simulink model "CHB_inverter_v2"  (R2025a)
settings: Solver=FixedStepDiscrete  StartTime=0.0  StopTime=T_stop  FixedStep=Ts  RelTol=1e-3
values from neighbouring files (symbols this model uses):
  Ts = Ts_pwr    (= 1e-06)    [init_microgrid.m]
  Vdc = sm(Vdc,100)    [make_figures.m]
undefined symbols (not defined in the file or in its folder): Cf, Lf, Rd, RLf, Rload
libraries: spsSeriesRLCBranchLib x3, spsUniversalBridgeLib x2, spsVoltageMeasurementLib x2, spsDCVoltageSourceLib x2, spsGroundLib x1, spsCurrentMeasurementLib x1, spspowerguiLib x1
settings Model: Creator=msssr  LastModifiedBy=msssr
settings DataIOCC: SignalLogging=off

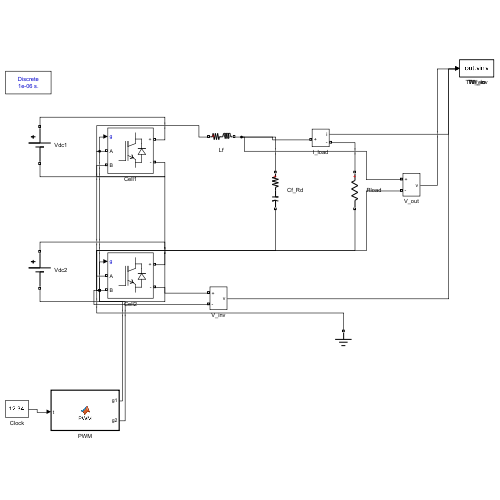
[thumbnail: Simulink's stored preview of the top-level diagram]
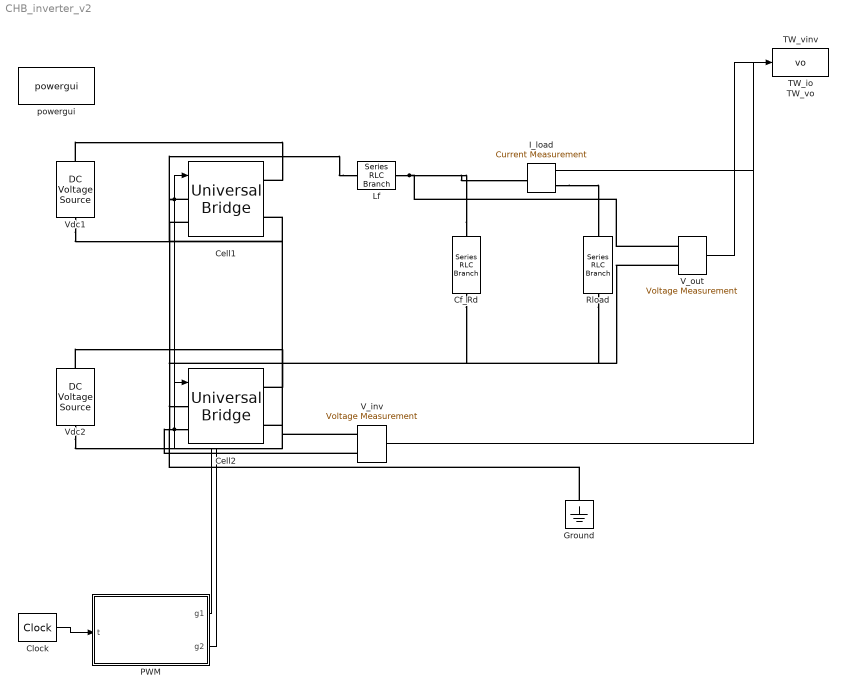
== system CHB_inverter_v2 ==
  Cell1 : spsUniversalBridgeLib/Universal Bridge  Arms=2  SnubberResistance=1e5  SnubberCapacitance=inf  Device=IGBT / Diodes  Ron=1e-3  Lon=0  ForwardVoltages="[  0  0  ]"  ForwardVoltage=0  GTOparameters=[ 10e-6 , 20e-6 ]  IGBTparameters=[ 1e-6 , 2e-6 ]  Measurements=None  Measurements_2=None  converterType=Rectifier
  Cell2 : spsUniversalBridgeLib/Universal Bridge  Arms=2  SnubberResistance=1e5  SnubberCapacitance=inf  Device=IGBT / Diodes  Ron=1e-3  Lon=0  ForwardVoltages="[  0  0  ]"  ForwardVoltage=0  GTOparameters=[ 10e-6 , 20e-6 ]  IGBTparameters=[ 1e-6 , 2e-6 ]  Measurements=None  Measurements_2=None  converterType=Rectifier
  Cf_Rd : spsSeriesRLCBranchLib/Series RLC Branch  LConnTagsString=__new0  RConnTagsString=__new0  BranchType=RC  Resistance=max(Rd,1e-6)  Inductance=1e-3  SetiL0=off  InitialCurrent=0  Capacitance=Cf  Setx0=off  InitialVoltage=0  Measurements=None
  Clock : DigitalClock  SampleTime=Ts
  Ground : spsGroundLib/Ground  LConnTagsString=a
  I_load : spsCurrentMeasurementLib/Current Measurement  PhasorSimulation=off  OutputType=Complex  PSBequivalent=0
  Lf : spsSeriesRLCBranchLib/Series RLC Branch  LConnTagsString=__new0  RConnTagsString=__new0  BranchType=RL  Resistance=RLf  Inductance=Lf  SetiL0=off  InitialCurrent=0  Capacitance=1e-6  Setx0=off  InitialVoltage=0  Measurements=None
  PWM : MATLAB Function  TreatAsAtomicUnit=on
  Rload : spsSeriesRLCBranchLib/Series RLC Branch  LConnTagsString=__new0  RConnTagsString=__new0  BranchType=R  Resistance=Rload  Inductance=1e-3  SetiL0=off  InitialCurrent=0  Capacitance=1e-6  Setx0=off  InitialVoltage=0  Measurements=None
  TW_io : ToWorkspace  VariableName=io  SaveFormat=Structure With Time  SampleTime=-1
  TW_vinv : ToWorkspace  VariableName=vinv  SaveFormat=Structure With Time  SampleTime=-1
  TW_vo : ToWorkspace  VariableName=vo  SaveFormat=Structure With Time  SampleTime=-1
  V_inv : spsVoltageMeasurementLib/Voltage Measurement  PhasorSimulation=off  OutputType=Complex  PSBequivalent=0
  V_out : spsVoltageMeasurementLib/Voltage Measurement  PhasorSimulation=off  OutputType=Complex  PSBequivalent=0
  Vdc1 : spsDCVoltageSourceLib/DC Voltage Source  Amplitude=Vdc  Measurements=None
  Vdc2 : spsDCVoltageSourceLib/DC Voltage Source  Amplitude=Vdc  Measurements=None
  powergui : spspowerguiLib/powergui  Priority=1  SimulationMode=Discrete  SampleTime=Ts  frequency=60  Iterations=50  frequencyindice=60  Pbase=100e6  ErrMax=1e-4  UnitsV=kV  UnitsW=MW  buscounter=0  FunctionMessages=off  echomessages=off  EnableUseOfTLC=off  CurrentSourceSwitches=off  DisableSnubberDevices=off  DisableRonSwitches=off  DisableVfSwitches=off  DisplayEquations=off  AutomaticDiscreteSolvers=off  SolverType=Tustin/Backward Euler (TBE)  Interpol=off  ExternalGateDelay=off  methode=off  Ts=100  x0status=blocks  SPID=on  SwTol=0  HookPort=off  NonlinearTolerance=1e-4  nMaxIteration=100  ContinueOnMaxIteration=off  RestoreLinks=warning  ResistiveCurrentMeasurement=off  Frange=[0:2:500]  Ylog=off  Xlog=on  ShowGrid=off  save=off  variable=ZData  structure=0  ZoomFFT=off  StartTime=0.0  cycles=1  DisplayStyle=1  fundamental=60  FreqAxis=off  MaxFrequency=1000  frequencyindicesteady=1  RmsSteady=1  display=off
  wires:
  Clock/1 -> PWM/1(t)
  PWM/1(g1) -> Cell1/1
  PWM/2(g2) -> Cell2/1
  V_out/1 -> TW_vo/1
  I_load/1 -> TW_io/1
  V_inv/1 -> TW_vinv/1
  connections:
  Vdc1/RConn1 -- Cell1/RConn1
  Vdc1/LConn1 -- Cell1/RConn2
  Vdc2/RConn1 -- Cell2/RConn1
  Vdc2/LConn1 -- Cell2/RConn2
  Cell1/LConn2 -- Cell2/LConn1
  Lf/LConn1 -- Cell1/LConn1 -- V_inv/LConn1
  Cf_Rd/LConn1 -- Lf/RConn1 -- I_load/LConn1 -- V_out/LConn1
  I_load/RConn1 -- Rload/LConn1
  Cf_Rd/RConn1 -- Rload/RConn1 -- Ground/LConn1 -- V_out/LConn2 -- Cell2/LConn2 -- V_inv/LConn2

== matlab function CHB_inverter_v2/PWM ==
  data: t input; g1 output; g2 output
function [g1, g2] = PWM(t)
% Unipolar phase-shifted carrier PWM, 2 cells, carriers 90 deg apart
ref = 0.8*sin(2*pi*50*t);
c1 = (2/pi)*asin(sin(2*pi*1000*t));
c2 = (2/pi)*asin(sin(2*pi*1000*t + pi/2));
a1 = double(ref > c1);  b1 = double(-ref > c1);
a2 = double(ref > c2);  b2 = double(-ref > c2);
g1 = [a1; 1-a1; b1; 1-b1];   % [upper A; lower A; upper B; lower B]
g2 = [a2; 1-a2; b2; 1-b2];
